simulink model "Grid_Forming_Inverters"  (R2024b)
settings: Solver=VariableStepAuto  StartTime=0.0  StopTime=GFM_Sim.t_stop  RelTol=1e-3
InitFcn:
  | addpath(genpath(fullfile(fileparts(fileparts(fileparts(get_param(bdroot,'FileName')))),'code','functions')));initialize_equipment_model_from_callback(bdroot);
undefined symbols (not defined in the file): Cf, f, GFM_CL, GFM_Droop, GFM_VI, GFM_VL, I_base_peak, L1, L2, Lg, R_C, R_L1, R_L2, Rg, S_base, V_base_phase, V_in, Vg
libraries: slpidlib x4, spsabctodq0Lib x4, spsThreePhaseSeriesRLCBranchLib x4, spsControlledVoltageSourceLib x3, spsCurrentMeasurementLib x3, spsVoltageMeasurementLib x3, spsGroundLib x2, spsThreePhaseVIMeasurementLib x2, spsdq0toabcLib x1, simulink x1, spsThreePhaseBreakerLib x1, spsThreePhaseProgrammableVoltageSourceLib x1
settings Model: Creator=ANYE  LastModifiedBy=AnYe
settings SolverCC: ZeroCrossAlgorithm=Adaptive
settings OptimizationCC: ReuseModelBlockBuffer=off
settings DebuggingCC: AlgebraicLoopMsg=none  IgnoredZcDiagnostic=none
settings RTWCC: GPUComputeCapability=3.5

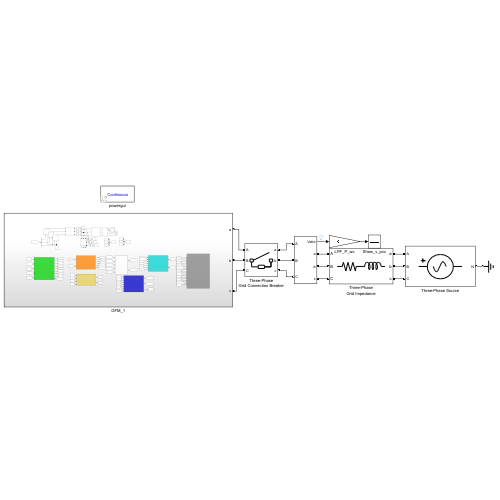
[thumbnail: Simulink's stored preview of the top-level diagram]
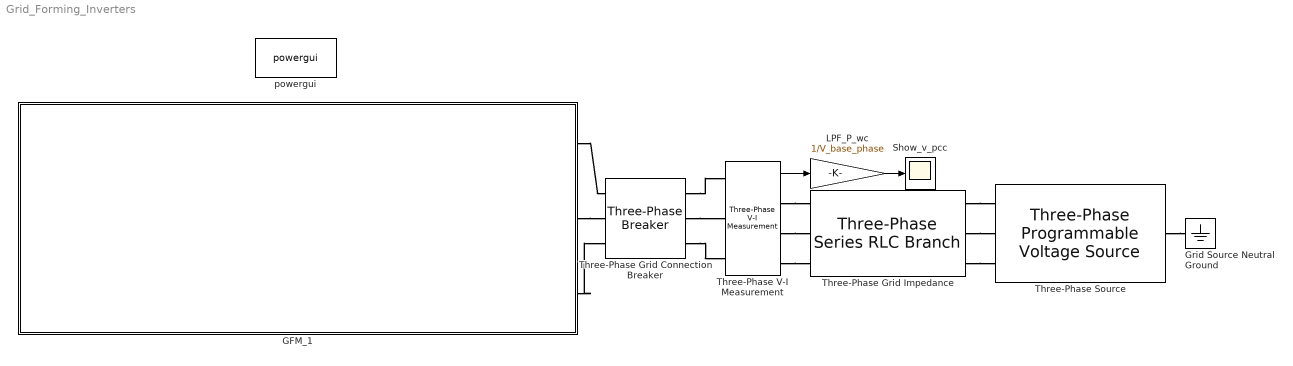
== system Grid_Forming_Inverters ==
  GFM_1 : Subsystem
  Grid Source Neutral Ground : spsGroundLib/Ground  LConnTagsString=a
  LPF_P_wc : Gain  Gain=1/V_base_phase
  Show_v_pcc : Scope
  Three-Phase Grid Connection Breaker : spsThreePhaseBreakerLib/Three-Phase Breaker  InitialState=open  SwitchA=on  SwitchB=on  SwitchC=on  SwitchTimes=t_close  External=off  BreakerResistance=0.01  SnubberResistance=1e6  SnubberCapacitance=inf  Measurements=None
  Three-Phase Grid Impedance : spsThreePhaseSeriesRLCBranchLib/Three-Phase Series RLC Branch  LConnTagsString=A|B|C  RConnTagsString=A|B|C  BranchType=RL  Resistance=Rg  Inductance=Lg  Capacitance=1e-6  Measurements=None
  Three-Phase V-I Measurement : spsThreePhaseVIMeasurementLib/Three-Phase V-I Measurement  VoltageMeasurement=phase-to-ground  SetLabelV=off  LabelV=Vabc  Vpu=off  VpuLL=off  CurrentMeasurement=no  SetLabelI=off  LabelI=Iabc  Ipu=off  Pbase=100e6  Vbase=500e3  OutputType=Complex  PhasorSimulation=off  PSBequivalent=0
  Three-Phase Source : spsThreePhaseProgrammableVoltageSourceLib/Three-Phase Programmable Voltage Source  PositiveSequence=[Vg 0 f]  VariationEntity=Amplitude  VariationType=Table of time-amplitude pairs  VariationTypeAlt=Step  VariationStep=0.5  VariationRate=10  VariationMagnitude=0.3  VariationFrequency=2  VariationTiming=[1 2]  VariationPhaseA=off  Amplitudes=GFM_GridSource.Amplitudes_pu  TimeValues=GFM_GridSource.TimeValues_s  HarmonicGeneration=off  HarmonicA=[3 0.2 -25 0]  HarmonicB=[2 0.15 35 2]  Timing="[0.05  3]"  BusType=swing  Pref=0  Qref=0  Qmin=-inf  Qmax=inf
  powergui : spspowerguiLib/powergui  Priority=1  SimulationMode=Continuous  SampleTime=50e-6  frequency=f  Iterations=50  frequencyindice=50  Pbase=100e6  ErrMax=1e-4  UnitsV=kV  UnitsW=MW  buscounter=0  FunctionMessages=off  echomessages=off  EnableUseOfTLC=off  CurrentSourceSwitches=off  DisableSnubberDevices=off  DisableRonSwitches=off  DisableVfSwitches=off  DisplayEquations=off  AutomaticDiscreteSolvers=off  SolverType=Tustin/Backward Euler (TBE)  Interpol=off  ExternalGateDelay=off  methode=off  Ts=100  x0status=blocks  SPID=on  SwTol=0  HookPort=off  NonlinearTolerance=1e-4  nMaxIteration=100  ContinueOnMaxIteration=off  RestoreLinks=warning  ResistiveCurrentMeasurement=off  Frange=[0:2:500]  Ylog=off  Xlog=on  ShowGrid=off  save=off  variable=ZData  structure=0  ZoomFFT=off  StartTime=0.0  cycles=1  DisplayStyle=1  fundamental=f  FreqAxis=off  MaxFrequency=1000  frequencyindicesteady=1  RmsSteady=1  display=off
  wires:
  Three-Phase V-I Measurement/1 -> LPF_P_wc/1
  LPF_P_wc/1 -> Show_v_pcc/1
  connections:
  Three-Phase V-I Measurement/RConn1 -- Three-Phase Grid Impedance/LConn1
  Three-Phase V-I Measurement/RConn2 -- Three-Phase Grid Impedance/LConn2
  Three-Phase V-I Measurement/RConn3 -- Three-Phase Grid Impedance/LConn3
  GFM_1/RConn1 -- Three-Phase Grid Connection Breaker/LConn1
  Three-Phase Grid Connection Breaker/RConn1 -- Three-Phase V-I Measurement/LConn1
  GFM_1/RConn2 -- Three-Phase Grid Connection Breaker/LConn2
  Three-Phase Grid Connection Breaker/RConn2 -- Three-Phase V-I Measurement/LConn2
  GFM_1/RConn3 -- Three-Phase Grid Connection Breaker/LConn3
  Three-Phase Grid Connection Breaker/RConn3 -- Three-Phase V-I Measurement/LConn3
  Three-Phase Grid Impedance/RConn1 -- Three-Phase Source/RConn1
  Three-Phase Grid Impedance/RConn2 -- Three-Phase Source/RConn2
  Three-Phase Grid Impedance/RConn3 -- Three-Phase Source/RConn3
  Three-Phase Source/LConn1 -- Grid Source Neutral Ground/LConn1

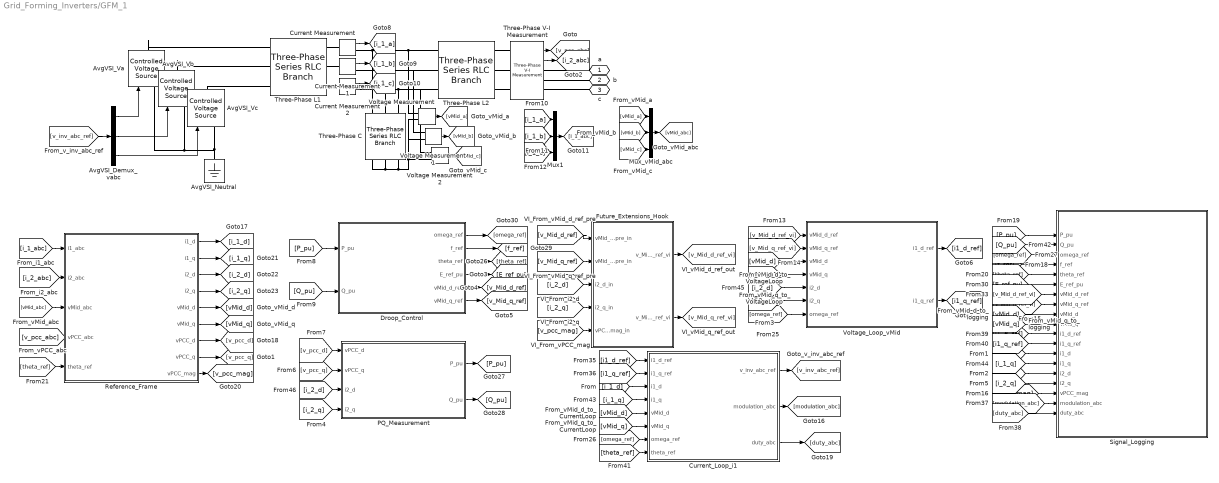
== system Grid_Forming_Inverters/GFM_1 ==
  AvgVSI_Demux_vabc : Demux  Outputs=3
  AvgVSI_Neutral : spsGroundLib/Ground  LConnTagsString=a
  AvgVSI_Va : spsControlledVoltageSourceLib/Controlled Voltage Source  Initialize=on  Source_Type=AC  Amplitude=0  Phase=0  Frequency=0  Measurements=None
  AvgVSI_Vb : spsControlledVoltageSourceLib/Controlled Voltage Source  Initialize=on  Source_Type=AC  Amplitude=0  Phase=0  Frequency=0  Measurements=None
  AvgVSI_Vc : spsControlledVoltageSourceLib/Controlled Voltage Source  Initialize=on  Source_Type=AC  Amplitude=0  Phase=0  Frequency=0  Measurements=None
  Current Measurement : spsCurrentMeasurementLib/Current Measurement  PhasorSimulation=off  OutputType=Complex  PSBequivalent=0
  Current Measurement1 : spsCurrentMeasurementLib/Current Measurement  PhasorSimulation=off  OutputType=Complex  PSBequivalent=0
  Current Measurement2 : spsCurrentMeasurementLib/Current Measurement  PhasorSimulation=off  OutputType=Complex  PSBequivalent=0
  Current_Loop_i1 : Subsystem
  Droop_Control : Subsystem
  Future_Extensions_Hook : Subsystem
      settings: AttributesFormatString=Unity pass-through in this version\nReserved: virtual impedance / LVRT / current limiting
  Mux1 : Mux  Inputs=3
  Mux_vMid_abc : Mux  Inputs=3
  PQ_Measurement : Subsystem
  Reference_Frame : Subsystem
  Signal_Logging : Subsystem
  Three-Phase C : spsThreePhaseSeriesRLCBranchLib/Three-Phase Series RLC Branch  LConnTagsString=A|B|C  RConnTagsString=A|B|C  BranchType=RC  Resistance=R_C  Inductance=1e-6  Capacitance=Cf  Measurements=None
  Three-Phase L1 : spsThreePhaseSeriesRLCBranchLib/Three-Phase Series RLC Branch  LConnTagsString=A|B|C  RConnTagsString=A|B|C  BranchType=RL  Resistance=R_L1  Inductance=L1  Capacitance=1e-6  Measurements=None
  Three-Phase L2 : spsThreePhaseSeriesRLCBranchLib/Three-Phase Series RLC Branch  LConnTagsString=A|B|C  RConnTagsString=A|B|C  BranchType=RL  Resistance=R_L2  Inductance=L2  Capacitance=1e-6  Measurements=None
  Three-Phase V-I Measurement : spsThreePhaseVIMeasurementLib/Three-Phase V-I Measurement  VoltageMeasurement=phase-to-ground  SetLabelV=off  LabelV=Vabc  Vpu=off  VpuLL=off  CurrentMeasurement=yes  SetLabelI=off  LabelI=Iabc  Ipu=off  Pbase=100e6  Vbase=500e3  OutputType=Complex  PhasorSimulation=off  PSBequivalent=0
  Voltage Measurement : spsVoltageMeasurementLib/Voltage Measurement  PhasorSimulation=off  OutputType=Complex  PSBequivalent=0
  Voltage Measurement1 : spsVoltageMeasurementLib/Voltage Measurement  PhasorSimulation=off  OutputType=Complex  PSBequivalent=0
  Voltage Measurement2 : spsVoltageMeasurementLib/Voltage Measurement  PhasorSimulation=off  OutputType=Complex  PSBequivalent=0
  Voltage_Loop_vMid : Subsystem
  a : PMIOPort  Side=Right
  b : PMIOPort  Port=2  Side=Right
  c : PMIOPort  Port=3  Side=Right
  wires:
  Three-Phase V-I Measurement/1 -> [v_pcc_abc]
  Current Measurement/1 -> [i_1_a]
  Current Measurement1/1 -> [i_1_b]
  Current Measurement2/1 -> [i_1_c]
  Voltage Measurement1/1 -> [vMid_b]
  Three-Phase V-I Measurement/2 -> [i_2_abc]
  Voltage Measurement2/1 -> [vMid_c]
  Voltage Measurement/1 -> [vMid_a]
  Mux_vMid_abc/1 -> [vMid_abc]
  Mux1/1 -> [i_1_abc]
  [i_1_c] -> Mux1/3
  [vMid_c] -> Mux_vMid_abc/3
  [vMid_b] -> Mux_vMid_abc/2
  [vMid_a] -> Mux_vMid_abc/1
  [i_1_a] -> Mux1/1
  [i_1_b] -> Mux1/2
  [v_inv_abc_ref] -> AvgVSI_Demux_vabc/1
  AvgVSI_Demux_vabc/1 -> AvgVSI_Va/1
  AvgVSI_Demux_vabc/2 -> AvgVSI_Vb/1
  AvgVSI_Demux_vabc/3 -> AvgVSI_Vc/1
  Current_Loop_i1/3(duty_abc) -> [duty_abc]
  Current_Loop_i1/2(modulation_abc) -> [modulation_abc]
  [i1_d_ref] -> Current_Loop_i1/1(i1_d_ref)
  [omega_ref] -> Current_Loop_i1/7(omega_ref)
  [duty_abc] -> Signal_Logging/19(duty_abc)
  PQ_Measurement/2(Q_pu) -> [Q_pu]
  [omega_ref] -> Voltage_Loop_vMid/7(omega_ref)
  [omega_ref] -> Signal_Logging/3(omega_ref)
  Reference_Frame/2(i1_q) -> [i_1_q]
  [Q_pu] -> Signal_Logging/2(Q_pu)
  [i_1_d] -> Current_Loop_i1/3(i1_d)
  Droop_Control/4(E_ref_pu) -> [E_ref_pu]
  Droop_Control/5(vMid_d_ref) -> [v_Mid_d_ref]
  [i_2_q] -> Voltage_Loop_vMid/6(i2_q)
  Reference_Frame/3(i2_d) -> [i_2_d]
  [vMid_d] -> Signal_Logging/9(vMid_d)
  [v_pcc_q] -> PQ_Measurement/2(vPCC_q)
  [P_pu] -> Signal_Logging/1(P_pu)
  [vMid_q] -> Signal_Logging/10(vMid_q)
  [v_Mid_d_ref_vi] -> Signal_Logging/7(vMid_d_ref)
  [i_2_d] -> PQ_Measurement/3(i2_d)
  [theta_ref] -> Current_Loop_i1/8(theta_ref)
  Reference_Frame/6(vMid_q) -> [vMid_q]
  [i_2_d] -> Signal_Logging/15(i2_d)
  [i1_d_ref] -> Signal_Logging/11(i1_d_ref)
  [i_1_q] -> Signal_Logging/14(i1_q)
  [E_ref_pu] -> Signal_Logging/6(E_ref_pu)
  [i_2_d] -> Voltage_Loop_vMid/5(i2_d)
  PQ_Measurement/1(P_pu) -> [P_pu]
  Droop_Control/3(theta_ref) -> [theta_ref]
  Reference_Frame/9(vPCC_mag) -> [v_pcc_mag]
  [f_ref] -> Signal_Logging/4(f_ref)
  [i_1_d] -> Signal_Logging/13(i1_d)
  Reference_Frame/7(vPCC_d) -> [v_pcc_d]
  Droop_Control/2(f_ref) -> [f_ref]
  [i_2_q] -> Signal_Logging/16(i2_q)
  [i_1_q] -> Current_Loop_i1/4(i1_q)
  [v_pcc_d] -> PQ_Measurement/1(vPCC_d)
  Reference_Frame/4(i2_q) -> [i_2_q]
  Droop_Control/1(omega_ref) -> [omega_ref]
  [i_2_q] -> PQ_Measurement/4(i2_q)
  [modulation_abc] -> Signal_Logging/18(modulation_abc)
  Reference_Frame/1(i1_d) -> [i_1_d]
  [i1_q_ref] -> Current_Loop_i1/2(i1_q_ref)
  [vMid_q] -> Voltage_Loop_vMid/4(vMid_q)
  [i1_q_ref] -> Signal_Logging/12(i1_q_ref)
  [vMid_d] -> Voltage_Loop_vMid/3(vMid_d)
  [P_pu] -> Droop_Control/1(P_pu)
  [Q_pu] -> Droop_Control/2(Q_pu)
  [theta_ref] -> Reference_Frame/5(theta_ref)
  [vMid_q] -> Current_Loop_i1/6(vMid_q)
  [vMid_d] -> Current_Loop_i1/5(vMid_d)
  Reference_Frame/5(vMid_d) -> [vMid_d]
  [v_pcc_mag] -> Signal_Logging/17(vPCC_mag)
  Reference_Frame/8(vPCC_q) -> [v_pcc_q]
  [theta_ref] -> Signal_Logging/5(theta_ref)
  Current_Loop_i1/1(v_inv_abc_ref) -> [v_inv_abc_ref]
  [i_1_abc] -> Reference_Frame/1(i1_abc)
  [i_2_abc] -> Reference_Frame/2(i2_abc)
  [vMid_abc] -> Reference_Frame/3(vMid_abc)
  [v_pcc_abc] -> Reference_Frame/4(vPCC_abc)
  [v_Mid_d_ref_vi] -> Voltage_Loop_vMid/1(vMid_d_ref)
  Droop_Control/6(vMid_q_ref) -> [v_Mid_q_ref]
  [v_Mid_q_ref_vi] -> Voltage_Loop_vMid/2(vMid_q_ref)
  [v_Mid_q_ref_vi] -> Signal_Logging/8(vMid_q_ref)
  [v_Mid_d_ref] -> Future_Extensions_Hook/1(vMid_d_ref_pre_in)
  [v_Mid_q_ref] -> Future_Extensions_Hook/2(vMid_q_ref_pre_in)
  [i_2_d] -> Future_Extensions_Hook/3(i2_d_in)
  [i_2_q] -> Future_Extensions_Hook/4(i2_q_in)
  Voltage_Loop_vMid/1(i1_d_ref) -> [i1_d_ref]
  Voltage_Loop_vMid/2(i1_q_ref) -> [i1_q_ref]
  Future_Extensions_Hook/2(v_Mid_q_ref_vi) -> [v_Mid_q_ref_vi]
  Future_Extensions_Hook/1(v_Mid_d_ref_vi) -> [v_Mid_d_ref_vi]
  [v_pcc_mag] -> Future_Extensions_Hook/5(vPCC_mag_in)
  connections:
  Current Measurement1/LConn1 -- Three-Phase L1/RConn2
  a/RConn1 -- Three-Phase V-I Measurement/RConn1
  Three-Phase C/RConn1 -- Voltage Measurement2/LConn2 -- Voltage Measurement1/LConn2 -- Voltage Measurement/LConn2 -- Three-Phase C/RConn3 -- Three-Phase C/RConn2
  Three-Phase C/LConn2 -- Three-Phase L2/LConn2 -- Voltage Measurement1/LConn1 -- Current Measurement1/RConn1
  Three-Phase C/LConn3 -- Three-Phase L2/LConn3 -- Voltage Measurement2/LConn1 -- Current Measurement2/RConn1
  Three-Phase V-I Measurement/LConn2 -- Three-Phase L2/RConn2
  Three-Phase C/LConn1 -- Current Measurement/RConn1 -- Three-Phase L2/LConn1 -- Voltage Measurement/LConn1
  Three-Phase L1/RConn3 -- Current Measurement2/LConn1
  Current Measurement/LConn1 -- Three-Phase L1/RConn1
  Three-Phase V-I Measurement/LConn3 -- Three-Phase L2/RConn3
  b/RConn1 -- Three-Phase V-I Measurement/RConn2
  Three-Phase V-I Measurement/LConn1 -- Three-Phase L2/RConn1
  c/RConn1 -- Three-Phase V-I Measurement/RConn3
  AvgVSI_Vb/RConn1 -- Three-Phase L1/LConn2
  AvgVSI_Va/RConn1 -- Three-Phase L1/LConn1
  Three-Phase L1/LConn3 -- AvgVSI_Vc/RConn1
  AvgVSI_Va/LConn1 -- AvgVSI_Vc/LConn1 -- AvgVSI_Neutral/LConn1 -- AvgVSI_Vb/LConn1

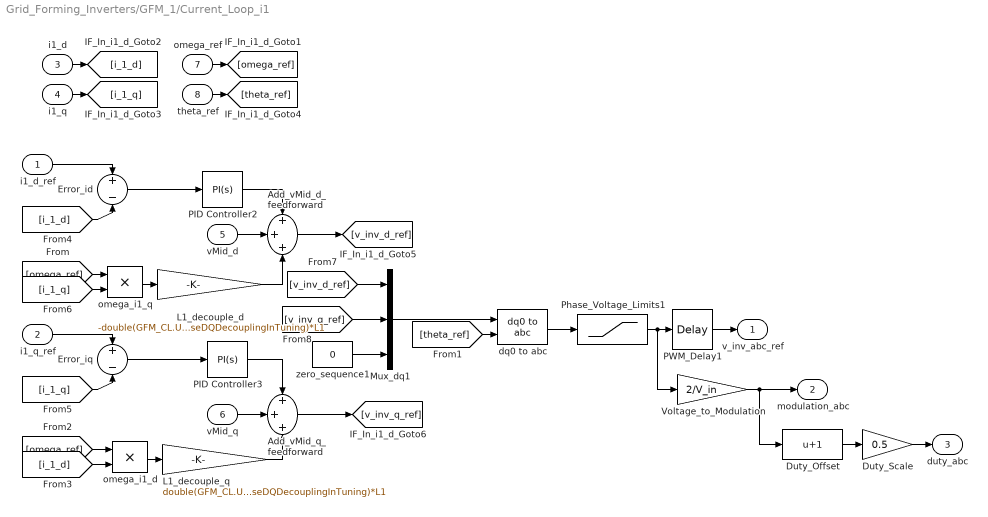
== system Grid_Forming_Inverters/GFM_1/Current_Loop_i1 ==
  i1_d_ref : Inport
  i1_q_ref : Inport  Port=2
  i1_d : Inport  Port=3
  i1_q : Inport  Port=4
  vMid_d : Inport  Port=5
  vMid_q : Inport  Port=6
  omega_ref : Inport  Port=7
  theta_ref : Inport  Port=8
  Add_vMid_d_feedforward : Sum  Inputs=+++
  Add_vMid_q_feedforward : Sum  Inputs=+++
  Duty_Offset : Bias  Bias=1  SaturateOnIntegerOverflow=off
  Duty_Scale : Gain  Gain=0.5
  Error_id : Sum  Inputs=+-
  Error_iq : Sum  Inputs=+-
  L1_decouple_d : Gain  Gain=-double(GFM_CL.UseDQDecouplingInTuning)*L1
  L1_decouple_q : Gain  Gain=double(GFM_CL.UseDQDecouplingInTuning)*L1
  Mux_dq1 : Mux  Inputs=3
  PID Controller2 : slpidlib/PID Controller  Controller=PI  Form=Parallel  TimeDomain=Continuous-time  UseExternalTs=off  SampleTime=-1  IntegratorMethod=Forward Euler  FilterMethod=Forward Euler  ControllerParametersSource=internal  P=GFM_CL.Kp  I=GFM_CL.Ki  UseKiTs=off  D=0  UseExternalDerivativeSource=off  N=100  UseFilter=on  TunerSelectOption=Transfer Function Based (PID Tuner App)  InitialConditionSource=internal  InitialConditionForIntegrator=0  InitialConditionForFilter=0  DifferentiatorICPrevScaledInput=0  ExternalReset=none  TrackingMode=off  Kt=1  LimitOutput=off  SatLimitsSource=internal  UpperSaturationLimit=inf  LowerSaturationLimit=-inf  LinearizeAsGain=on  AntiWindupMode=none  Kb=1  LimitIntegrator=off  UpperIntegratorSaturationLimit=inf  LowerIntegratorSaturationLimit=-inf  POutMin=[]  POutMax=[]  IOutMin=[]  IOutMax=[]  DOutMin=[]  DOutMax=[]  NOutMin=[]  NOutMax=[]  SumOutMin=[]  SumOutMax=[]  SaturationOutMin=[]  SaturationOutMax=[]  PParamMin=[]  PParamMax=[]  IParamMin=[]  IParamMax=[]  DParamMin=[]  DParamMax=[]  NParamMin=[]  NParamMax=[]  KbParamMin=[]  KbParamMax=[]  KtParamMin=[]  KtParamMax=[]  KbOutMin=[]  KbOutMax=[]  KtOutMin=[]  KtOutMax=[]  IntegratorOutMin=[]  IntegratorOutMax=[]  FilterOutMin=[]  FilterOutMax=[]  SumI1OutMin=[]  SumI1OutMax=[]  SumI2OutMin=[]  SumI2OutMax=[]  SumI3OutMin=[]  SumI3OutMax=[]  SumI4OutMin=[]  SumI4OutMax=[]  SumDOutMin=[]  SumDOutMax=[]  DifferentiatorOutMin=[]  DifferentiatorOutMax=[]  FilterDiffOutCoefMin=[]  FilterDiffOutCoefMax=[]  ReciprocalOutMin=[]  ReciprocalOutMax=[]  SumDenOutMin=[]  SumDenOutMax=[]  SumNumOutMin=[]  SumNumOutMax=[]  DivideOutMin=[]  DivideOutMax=[]  UdiffTsProdOutMin=[]  UdiffTsProdOutMax=[]  NTsProdOutMin=[]  NTsProdOutMax=[]  UintegralTsProdOutMin=[]  UintegralTsProdOutMax=[]  UngainTsProdOutMin=[]  UngainTsProdOutMax=[]  ClampingZeroOutDataTypeStr=Inherit: Inherit via back propagation  ClampingZeroOutMin=[]  ClampingZeroOutMax=[]  FilterDenConstantOutDataTypeStr=Inherit: Inherit via back propagation  FilterDenConstantOutMin=[]  FilterDenConstantOutMax=[]  PCopyOutDataTypeStr=Inherit: Inherit via back propagation  PCopyOutMin=[]  PCopyOutMax=[]  NCopyOutDataTypeStr=Inherit: Inherit via back propagation  NCopyOutMin=[]  NCopyOutMax=[]  IntegratorContinuousStateAttributes=''  IntegratorStateMustResolveToSignalObject=off  IntegratorRTWStateStorageClass=Auto  FilterContinuousStateAttributes=''  FilterStateMustResolveToSignalObject=off  FilterRTWStateStorageClass=Auto  ParallelPVariant=InternalParameters  IdealPVariant=Disabled  IVariant=InternalParameters  DVariant=Disabled  IntegratorVariant=Continuous  SatVariant=Disabled  AWVariant=Passthrough  PCopyVariant=Disabled  TRVariant=Disabled  FdbkBlocksVariant=Forward  IdealPFdbkVariant=Disabled  SatFdbkVariant=Disabled  DerivativeFilterVariant=Disabled  NVariant=Disabled  NCopyVariant=Disabled_SignalSpec  FilterICVariant=Disabled  IntegratorICVariant=InternalICs  ExternalResetVariant=Disabled  TRSumVariant=Passthrough  SumFdbkVariant=Disabled  SumVariant=Sum_PI  TsampFilterVariant=InternalTs  TsampNgainVariant=Passthrough  TsampIntegralVariant=Disabled_SignalSpec  ExternalSaturationOutDataTypeStr=Inherit: Same as second input  DerivativeSourceVariant=Disabled  PreIntVariant=InternalPreInt
  PID Controller3 : slpidlib/PID Controller  Controller=PI  Form=Parallel  TimeDomain=Continuous-time  UseExternalTs=off  SampleTime=-1  IntegratorMethod=Forward Euler  FilterMethod=Forward Euler  ControllerParametersSource=internal  P=GFM_CL.Kp  I=GFM_CL.Ki  UseKiTs=off  D=0  UseExternalDerivativeSource=off  N=100  UseFilter=on  TunerSelectOption=Transfer Function Based (PID Tuner App)  InitialConditionSource=internal  InitialConditionForIntegrator=0  InitialConditionForFilter=0  DifferentiatorICPrevScaledInput=0  ExternalReset=none  TrackingMode=off  Kt=1  LimitOutput=off  SatLimitsSource=internal  UpperSaturationLimit=inf  LowerSaturationLimit=-inf  LinearizeAsGain=on  AntiWindupMode=none  Kb=1  LimitIntegrator=off  UpperIntegratorSaturationLimit=inf  LowerIntegratorSaturationLimit=-inf  POutMin=[]  POutMax=[]  IOutMin=[]  IOutMax=[]  DOutMin=[]  DOutMax=[]  NOutMin=[]  NOutMax=[]  SumOutMin=[]  SumOutMax=[]  SaturationOutMin=[]  SaturationOutMax=[]  PParamMin=[]  PParamMax=[]  IParamMin=[]  IParamMax=[]  DParamMin=[]  DParamMax=[]  NParamMin=[]  NParamMax=[]  KbParamMin=[]  KbParamMax=[]  KtParamMin=[]  KtParamMax=[]  KbOutMin=[]  KbOutMax=[]  KtOutMin=[]  KtOutMax=[]  IntegratorOutMin=[]  IntegratorOutMax=[]  FilterOutMin=[]  FilterOutMax=[]  SumI1OutMin=[]  SumI1OutMax=[]  SumI2OutMin=[]  SumI2OutMax=[]  SumI3OutMin=[]  SumI3OutMax=[]  SumI4OutMin=[]  SumI4OutMax=[]  SumDOutMin=[]  SumDOutMax=[]  DifferentiatorOutMin=[]  DifferentiatorOutMax=[]  FilterDiffOutCoefMin=[]  FilterDiffOutCoefMax=[]  ReciprocalOutMin=[]  ReciprocalOutMax=[]  SumDenOutMin=[]  SumDenOutMax=[]  SumNumOutMin=[]  SumNumOutMax=[]  DivideOutMin=[]  DivideOutMax=[]  UdiffTsProdOutMin=[]  UdiffTsProdOutMax=[]  NTsProdOutMin=[]  NTsProdOutMax=[]  UintegralTsProdOutMin=[]  UintegralTsProdOutMax=[]  UngainTsProdOutMin=[]  UngainTsProdOutMax=[]  ClampingZeroOutDataTypeStr=Inherit: Inherit via back propagation  ClampingZeroOutMin=[]  ClampingZeroOutMax=[]  FilterDenConstantOutDataTypeStr=Inherit: Inherit via back propagation  FilterDenConstantOutMin=[]  FilterDenConstantOutMax=[]  PCopyOutDataTypeStr=Inherit: Inherit via back propagation  PCopyOutMin=[]  PCopyOutMax=[]  NCopyOutDataTypeStr=Inherit: Inherit via back propagation  NCopyOutMin=[]  NCopyOutMax=[]  IntegratorContinuousStateAttributes=''  IntegratorStateMustResolveToSignalObject=off  IntegratorRTWStateStorageClass=Auto  FilterContinuousStateAttributes=''  FilterStateMustResolveToSignalObject=off  FilterRTWStateStorageClass=Auto  ParallelPVariant=InternalParameters  IdealPVariant=Disabled  IVariant=InternalParameters  DVariant=Disabled  IntegratorVariant=Continuous  SatVariant=Disabled  AWVariant=Passthrough  PCopyVariant=Disabled  TRVariant=Disabled  FdbkBlocksVariant=Forward  IdealPFdbkVariant=Disabled  SatFdbkVariant=Disabled  DerivativeFilterVariant=Disabled  NVariant=Disabled  NCopyVariant=Disabled_SignalSpec  FilterICVariant=Disabled  IntegratorICVariant=InternalICs  ExternalResetVariant=Disabled  TRSumVariant=Passthrough  SumFdbkVariant=Disabled  SumVariant=Sum_PI  TsampFilterVariant=InternalTs  TsampNgainVariant=Passthrough  TsampIntegralVariant=Disabled_SignalSpec  ExternalSaturationOutDataTypeStr=Inherit: Same as second input  DerivativeSourceVariant=Disabled  PreIntVariant=InternalPreInt
  PWM_Delay1 : TransportDelay  DelayTime=GFM_CL.PWMDelay
  Phase_Voltage_Limits1 : Saturate  UpperLimit=V_in/2  LowerLimit=-V_in/2
  Voltage_to_Modulation : Gain  Gain=2/V_in
  dq0 to abc : spsdq0toabcLib/dq0 to abc  Alignment=Aligned with phase A axis
  omega_i1_d : Product
  omega_i1_q : Product
  zero_sequence1 : Constant  Value=0
  v_inv_abc_ref : Outport
  modulation_abc : Outport  Port=2
  duty_abc : Outport  Port=3
  wires:
  i1_d_ref/1 -> Error_id/1
  i1_q_ref/1 -> Error_iq/1
  omega_i1_q/1 -> L1_decouple_d/1
  omega_i1_d/1 -> L1_decouple_q/1
  vMid_d/1 -> Add_vMid_d_feedforward/2
  L1_decouple_d/1 -> Add_vMid_d_feedforward/3
  vMid_q/1 -> Add_vMid_q_feedforward/2
  L1_decouple_q/1 -> Add_vMid_q_feedforward/3
  Add_vMid_d_feedforward/1 -> [v_inv_d_ref]
  Add_vMid_q_feedforward/1 -> [v_inv_q_ref]
  omega_ref/1 -> [omega_ref]
  [omega_ref] -> omega_i1_q/1
  [omega_ref] -> omega_i1_d/1
  [i_1_d] -> omega_i1_d/2
  i1_d/1 -> [i_1_d]
  [i_1_d] -> Error_id/2
  i1_q/1 -> [i_1_q]
  [i_1_q] -> Error_iq/2
  [i_1_q] -> omega_i1_q/2
  PID Controller2/1 -> Add_vMid_d_feedforward/1
  Error_id/1 -> PID Controller2/1
  Error_iq/1 -> PID Controller3/1
  PID Controller3/1 -> Add_vMid_q_feedforward/1
  [theta_ref] -> dq0 to abc/2
  theta_ref/1 -> [theta_ref]
  Mux_dq1/1 -> dq0 to abc/1
  zero_sequence1/1 -> Mux_dq1/3
  [v_inv_q_ref] -> Mux_dq1/2
  [v_inv_d_ref] -> Mux_dq1/1
  Phase_Voltage_Limits1/1 -> Voltage_to_Modulation/1, PWM_Delay1/1
  dq0 to abc/1 -> Phase_Voltage_Limits1/1
  PWM_Delay1/1 -> v_inv_abc_ref/1
  Duty_Offset/1 -> Duty_Scale/1
  Duty_Scale/1 -> duty_abc/1
  Voltage_to_Modulation/1 -> modulation_abc/1, Duty_Offset/1

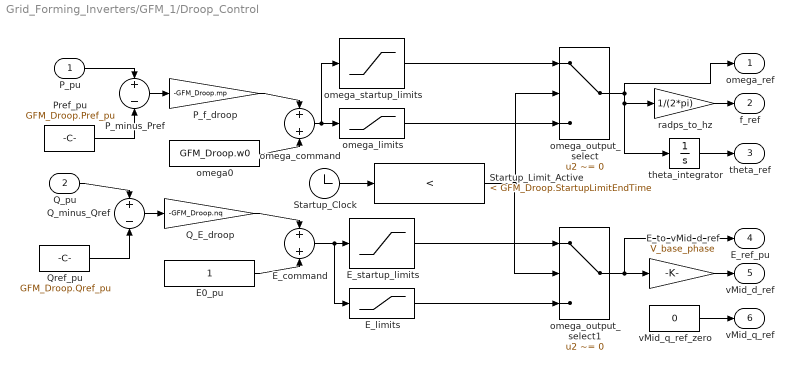
== system Grid_Forming_Inverters/GFM_1/Droop_Control ==
  P_pu : Inport
  Q_pu : Inport  Port=2
  E0_pu : Constant
  E_command : Sum
  E_limits : Saturate  UpperLimit=GFM_Droop.E_max_pu  LowerLimit=GFM_Droop.E_min_pu
  E_startup_limits : Saturate  UpperLimit=GFM_Droop.Startup_E_max_pu  LowerLimit=GFM_Droop.Startup_E_min_pu
  E_to_vMid_d_ref : Gain  Gain=V_base_phase
  P_f_droop : Gain  Gain=-GFM_Droop.mp
  P_minus_Pref : Sum  Inputs=+-
  Pref_pu : Constant  Value=GFM_Droop.Pref_pu
  Q_E_droop : Gain  Gain=-GFM_Droop.nq
  Q_minus_Qref : Sum  Inputs=+-
  Qref_pu : Constant  Value=GFM_Droop.Qref_pu
  Startup_Clock : Clock
  Startup_Limit_Active : simulink/Logic and Bit Operations/Compare To Constant  relop=<  const=GFM_Droop.StartupLimitEndTime  OutDataTypeStr=boolean
  omega0 : Constant  Value=GFM_Droop.w0
  omega_command : Sum
  omega_limits : Saturate  UpperLimit=GFM_Droop.w_max  LowerLimit=GFM_Droop.w_min
  omega_output_select : Switch  Criteria=u2 ~= 0  SaturateOnIntegerOverflow=off  InputSameDT=off
  omega_output_select1 : Switch  Criteria=u2 ~= 0  SaturateOnIntegerOverflow=off  InputSameDT=off
  omega_startup_limits : Saturate  UpperLimit=GFM_Droop.Startup_w_max  LowerLimit=GFM_Droop.Startup_w_min
  radps_to_hz : Gain  Gain=1/(2*pi)
  theta_integrator : Integrator  InitialCondition=GFM_Droop.theta0
  vMid_q_ref_zero : Constant  Value=0
  omega_ref : Outport
  f_ref : Outport  Port=2
  theta_ref : Outport  Port=3
  E_ref_pu : Outport  Port=4
  vMid_d_ref : Outport  Port=5
  vMid_q_ref : Outport  Port=6
  wires:
  P_pu/1 -> P_minus_Pref/1
  Pref_pu/1 -> P_minus_Pref/2
  P_minus_Pref/1 -> P_f_droop/1
  P_f_droop/1 -> omega_command/1
  omega0/1 -> omega_command/2
  omega_command/1 -> omega_limits/1, omega_startup_limits/1
  radps_to_hz/1 -> f_ref/1
  theta_integrator/1 -> theta_ref/1
  Q_pu/1 -> Q_minus_Qref/1
  Qref_pu/1 -> Q_minus_Qref/2
  Q_minus_Qref/1 -> Q_E_droop/1
  Q_E_droop/1 -> E_command/1
  E0_pu/1 -> E_command/2
  E_command/1 -> E_limits/1, E_startup_limits/1
  E_to_vMid_d_ref/1 -> vMid_d_ref/1
  vMid_q_ref_zero/1 -> vMid_q_ref/1
  omega_limits/1 -> omega_output_select/3
  omega_startup_limits/1 -> omega_output_select/1
  omega_output_select/1 -> radps_to_hz/1, theta_integrator/1, omega_ref/1
  Startup_Clock/1 -> Startup_Limit_Active/1
  Startup_Limit_Active/1 -> omega_output_select1/2, omega_output_select/2
  E_limits/1 -> omega_output_select1/3
  E_startup_limits/1 -> omega_output_select1/1
  omega_output_select1/1 -> E_to_vMid_d_ref/1, E_ref_pu/1

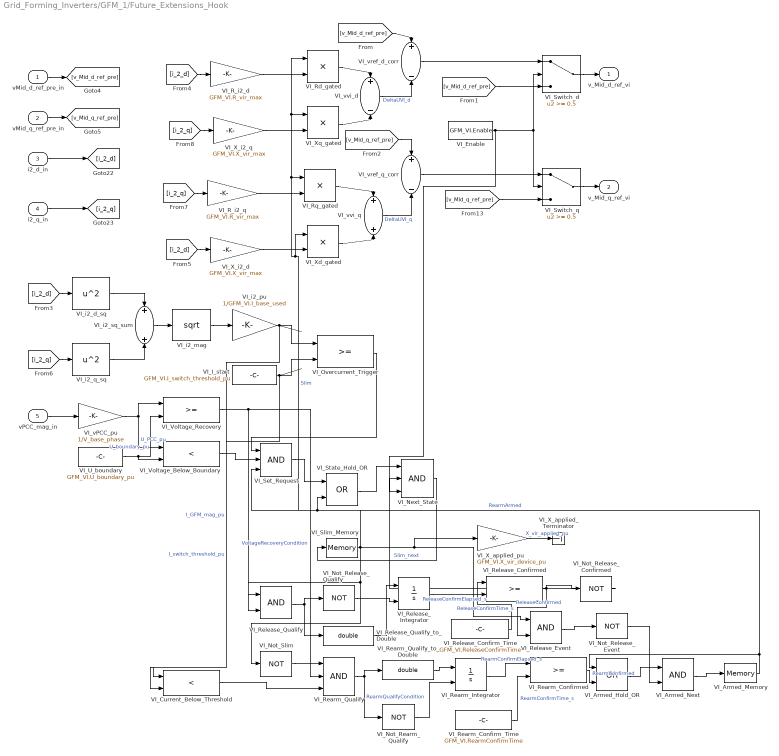
== system Grid_Forming_Inverters/GFM_1/Future_Extensions_Hook ==
  vMid_d_ref_pre_in : Inport
  vMid_q_ref_pre_in : Inport  Port=2
  i2_d_in : Inport  Port=3
  i2_q_in : Inport  Port=4
  vPCC_mag_in : Inport  Port=5
  VI_Armed_Hold_OR : Logic  Operator=OR  AllPortsSameDT=off  OutDataTypeStr=boolean
  VI_Armed_Memory : Memory  InitialCondition=1
  VI_Armed_Next : Logic  AllPortsSameDT=off  OutDataTypeStr=boolean
  VI_Current_Below_Threshold : RelationalOperator  Operator=<  OutDataTypeStr=boolean  RndMeth=Simplest  InputSameDT=off
  VI_Enable : Constant  Value=GFM_VI.Enable
  VI_I_start : Constant  Value=GFM_VI.I_switch_threshold_pu
  VI_Next_State : Logic  Inputs=3  AllPortsSameDT=off  OutDataTypeStr=boolean
  VI_Not_Rearm_Qualify : Logic  Operator=NOT  AllPortsSameDT=off  OutDataTypeStr=boolean
  VI_Not_Release_Confirmed : Logic  Operator=NOT  AllPortsSameDT=off  OutDataTypeStr=boolean
  VI_Not_Release_Event : Logic  Operator=NOT  AllPortsSameDT=off  OutDataTypeStr=boolean
  VI_Not_Release_Qualify : Logic  Operator=NOT  AllPortsSameDT=off  OutDataTypeStr=boolean
  VI_Not_Slim : Logic  Operator=NOT  AllPortsSameDT=off  OutDataTypeStr=boolean
  VI_Overcurrent_Trigger : RelationalOperator  OutDataTypeStr=boolean  RndMeth=Simplest  InputSameDT=off
  VI_R_i2_d : Gain  Gain=GFM_VI.R_vir_max
  VI_R_i2_q : Gain  Gain=GFM_VI.R_vir_max
  VI_Rd_gated : Product  Inputs=**
  VI_Rearm_Confirm_Time : Constant  Value=GFM_VI.RearmConfirmTime
  VI_Rearm_Confirmed : RelationalOperator  OutDataTypeStr=boolean  RndMeth=Simplest  InputSameDT=off
  VI_Rearm_Integrator : Integrator  ExternalReset=level  LimitOutput=on  UpperSaturationLimit=GFM_VI.RearmConfirmTime  LowerSaturationLimit=0
  VI_Rearm_Qualify : Logic  Inputs=3  AllPortsSameDT=off  OutDataTypeStr=boolean
  VI_Rearm_Qualify_to_Double : DataTypeConversion  OutDataTypeStr=double  SaturateOnIntegerOverflow=off  RndMeth=Floor
  VI_Release_Confirm_Time : Constant  Value=GFM_VI.ReleaseConfirmTime
  VI_Release_Confirmed : RelationalOperator  OutDataTypeStr=boolean  RndMeth=Simplest  InputSameDT=off
  VI_Release_Event : Logic  AllPortsSameDT=off  OutDataTypeStr=boolean
  VI_Release_Integrator : Integrator  ExternalReset=level  LimitOutput=on  UpperSaturationLimit=GFM_VI.ReleaseConfirmTime  LowerSaturationLimit=0
  VI_Release_Qualify : Logic  AllPortsSameDT=off  OutDataTypeStr=boolean
  VI_Release_Qualify_to_Double : DataTypeConversion  OutDataTypeStr=double  SaturateOnIntegerOverflow=off  RndMeth=Floor
  VI_Rq_gated : Product  Inputs=**
  VI_Set_Request : Logic  Inputs=3  AllPortsSameDT=off  OutDataTypeStr=boolean
  VI_Slim_Memory : Memory
  VI_State_Hold_OR : Logic  Operator=OR  AllPortsSameDT=off  OutDataTypeStr=boolean
  VI_Switch_d : Switch  Threshold=0.5  SaturateOnIntegerOverflow=off  InputSameDT=off
  VI_Switch_q : Switch  Threshold=0.5  SaturateOnIntegerOverflow=off  InputSameDT=off
  VI_U_boundary : Constant  Value=GFM_VI.U_boundary_pu
  VI_Voltage_Below_Boundary : RelationalOperator  Operator=<  OutDataTypeStr=boolean  RndMeth=Simplest  InputSameDT=off
  VI_Voltage_Recovery : RelationalOperator  OutDataTypeStr=boolean  RndMeth=Simplest  InputSameDT=off
  VI_X_applied_Terminator : Terminator
  VI_X_applied_pu : Gain  Gain=GFM_VI.X_vir_device_pu  ParamDataTypeStr=double  OutDataTypeStr=double
  VI_X_i2_d : Gain  Gain=GFM_VI.X_vir_max
  VI_X_i2_q : Gain  Gain=GFM_VI.X_vir_max
  VI_Xd_gated : Product  Inputs=**
  VI_Xq_gated : Product  Inputs=**
  VI_i2_d_sq : Math  Operator=square
  VI_i2_mag : Math  Operator=sqrt
  VI_i2_pu : Gain  Gain=1/GFM_VI.I_base_used
  VI_i2_q_sq : Math  Operator=square
  VI_i2_sq_sum : Sum
  VI_vPCC_pu : Gain  Gain=1/V_base_phase
  VI_vref_d_corr : Sum  Inputs=+-
  VI_vref_q_corr : Sum  Inputs=+-
  VI_vvi_d : Sum  Inputs=+-
  VI_vvi_q : Sum
  v_Mid_d_ref_vi : Outport
  v_Mid_q_ref_vi : Outport  Port=2
  wires:
  VI_i2_d_sq/1 -> VI_i2_sq_sum/1
  VI_i2_q_sq/1 -> VI_i2_sq_sum/2
  VI_i2_sq_sum/1 -> VI_i2_mag/1
  VI_i2_mag/1 -> VI_i2_pu/1
  VI_i2_pu/1 -> VI_Overcurrent_Trigger/1, VI_Current_Below_Threshold/1  "I_GFM_mag_pu"
  VI_I_start/1 -> VI_Overcurrent_Trigger/2, VI_Current_Below_Threshold/2  "I_switch_threshold_pu"
  ? -> ?
  VI_R_i2_d/1 -> VI_Rd_gated/2
  VI_R_i2_q/1 -> VI_Rq_gated/2
  VI_X_i2_d/1 -> VI_Xd_gated/2
  VI_X_i2_q/1 -> VI_Xq_gated/2
  VI_Rd_gated/1 -> VI_vvi_d/1
  VI_Xq_gated/1 -> VI_vvi_d/2
  VI_Rq_gated/1 -> VI_vvi_q/1
  VI_Xd_gated/1 -> VI_vvi_q/2
  VI_vvi_d/1 -> VI_vref_d_corr/2  "DeltaUVI_d"
  VI_vvi_q/1 -> VI_vref_q_corr/2  "DeltaUVI_q"
  VI_vref_d_corr/1 -> VI_Switch_d/1
  VI_Enable/1 -> VI_Switch_d/2, VI_Switch_q/2, VI_Next_State/3
  VI_vref_q_corr/1 -> VI_Switch_q/1
  VI_Switch_d/1 -> v_Mid_d_ref_vi/1
  VI_Switch_q/1 -> v_Mid_q_ref_vi/1
  vMid_d_ref_pre_in/1 -> [v_Mid_d_ref_pre]
  [v_Mid_d_ref_pre] -> VI_vref_d_corr/1
  [v_Mid_d_ref_pre] -> VI_Switch_d/3
  vMid_q_ref_pre_in/1 -> [v_Mid_q_ref_pre]
  [v_Mid_q_ref_pre] -> VI_vref_q_corr/1
  i2_d_in/1 -> [i_2_d]
  [i_2_d] -> VI_i2_d_sq/1
  [i_2_d] -> VI_R_i2_d/1
  [i_2_d] -> VI_X_i2_d/1
  i2_q_in/1 -> [i_2_q]
  [i_2_q] -> VI_i2_q_sq/1
  [i_2_q] -> VI_X_i2_q/1
  [i_2_q] -> VI_R_i2_q/1
  [v_Mid_q_ref_pre] -> VI_Switch_q/3
  vPCC_mag_in/1 -> VI_vPCC_pu/1
  VI_vPCC_pu/1 -> VI_Voltage_Recovery/1, VI_Voltage_Below_Boundary/1  "U_PCC_pu"
  VI_U_boundary/1 -> VI_Voltage_Recovery/2, VI_Voltage_Below_Boundary/2  "U_boundary_pu"
  VI_Overcurrent_Trigger/1 -> VI_Set_Request/1
  VI_Voltage_Below_Boundary/1 -> VI_Set_Request/2
  VI_Set_Request/1 -> VI_State_Hold_OR/1
  VI_Slim_Memory/1 -> VI_Release_Qualify/2, VI_Not_Slim/1, VI_X_applied_pu/1, VI_Release_Event/1, VI_Rd_gated/1, VI_Xq_gated/1, VI_Rq_gated/1, VI_Xd_gated/1, VI_State_Hold_OR/2  "Slim"
  VI_State_Hold_OR/1 -> VI_Next_State/1
  VI_Not_Release_Confirmed/1 -> VI_Next_State/2
  VI_X_applied_pu/1 -> VI_X_applied_Terminator/1  "X_vir_applied_pu"
  VI_Next_State/1 -> VI_Slim_Memory/1  "Slim_next"
  VI_Voltage_Recovery/1 -> VI_Release_Qualify/1, VI_Rearm_Qualify/2  "VoltageRecoveryCondition"
  VI_Release_Qualify/1 -> VI_Release_Qualify_to_Double/1, VI_Not_Release_Qualify/1
  VI_Release_Qualify_to_Double/1 -> VI_Release_Integrator/1
  VI_Not_Release_Qualify/1 -> VI_Release_Integrator/2
  VI_Release_Integrator/1 -> VI_Release_Confirmed/1  "ReleaseConfirmElapsed_s"
  VI_Release_Confirm_Time/1 -> VI_Release_Confirmed/2  "ReleaseConfirmTime_s"
  VI_Release_Confirmed/1 -> VI_Not_Release_Confirmed/1, VI_Release_Event/2  "ReleaseConfirmed"
  VI_Not_Slim/1 -> VI_Rearm_Qualify/1
  VI_Current_Below_Threshold/1 -> VI_Rearm_Qualify/3
  VI_Rearm_Qualify/1 -> VI_Rearm_Qualify_to_Double/1, VI_Not_Rearm_Qualify/1  "RearmQualifyCondition"
  VI_Rearm_Qualify_to_Double/1 -> VI_Rearm_Integrator/1
  VI_Not_Rearm_Qualify/1 -> VI_Rearm_Integrator/2
  VI_Rearm_Integrator/1 -> VI_Rearm_Confirmed/1  "RearmConfirmElapsed_s"
  VI_Rearm_Confirm_Time/1 -> VI_Rearm_Confirmed/2  "RearmConfirmTime_s"
  VI_Release_Event/1 -> VI_Not_Release_Event/1
  VI_Armed_Memory/1 -> VI_Armed_Hold_OR/1, VI_Set_Request/3  "RearmArmed"
  VI_Rearm_Confirmed/1 -> VI_Armed_Hold_OR/2  "RearmConfirmed"
  VI_Armed_Hold_OR/1 -> VI_Armed_Next/1
  VI_Not_Release_Event/1 -> VI_Armed_Next/2
  VI_Armed_Next/1 -> VI_Armed_Memory/1

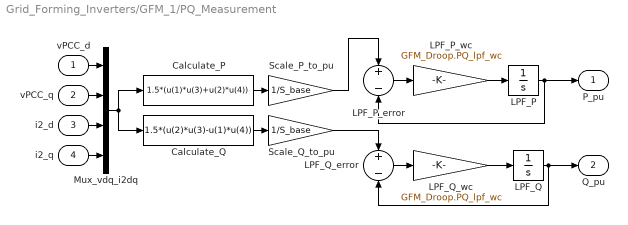
== system Grid_Forming_Inverters/GFM_1/PQ_Measurement ==
  vPCC_d : Inport
  vPCC_q : Inport  Port=2
  i2_d : Inport  Port=3
  i2_q : Inport  Port=4
  Calculate_P : Fcn  Expr=1.5*(u(1)*u(3)+u(2)*u(4))
  Calculate_Q : Fcn  Expr=1.5*(u(2)*u(3)-u(1)*u(4))
  LPF_P : Integrator  InitialCondition=GFM_Droop.Pref_pu
  LPF_P_error : Sum  Inputs=+-
  LPF_P_wc : Gain  Gain=GFM_Droop.PQ_lpf_wc
  LPF_Q : Integrator  InitialCondition=GFM_Droop.Qref_pu
  LPF_Q_error : Sum  Inputs=+-
  LPF_Q_wc : Gain  Gain=GFM_Droop.PQ_lpf_wc
  Mux_vdq_i2dq : Mux
  Scale_P_to_pu : Gain  Gain=1/S_base
  Scale_Q_to_pu : Gain  Gain=1/S_base
  P_pu : Outport
  Q_pu : Outport  Port=2
  wires:
  vPCC_d/1 -> Mux_vdq_i2dq/1
  vPCC_q/1 -> Mux_vdq_i2dq/2
  i2_d/1 -> Mux_vdq_i2dq/3
  i2_q/1 -> Mux_vdq_i2dq/4
  Mux_vdq_i2dq/1 -> Calculate_P/1, Calculate_Q/1
  Calculate_P/1 -> Scale_P_to_pu/1
  Scale_P_to_pu/1 -> LPF_P_error/1
  LPF_P/1 -> P_pu/1, LPF_P_error/2
  LPF_P_error/1 -> LPF_P_wc/1
  LPF_P_wc/1 -> LPF_P/1
  Calculate_Q/1 -> Scale_Q_to_pu/1
  Scale_Q_to_pu/1 -> LPF_Q_error/1
  LPF_Q/1 -> LPF_Q_error/2, Q_pu/1
  LPF_Q_error/1 -> LPF_Q_wc/1
  LPF_Q_wc/1 -> LPF_Q/1

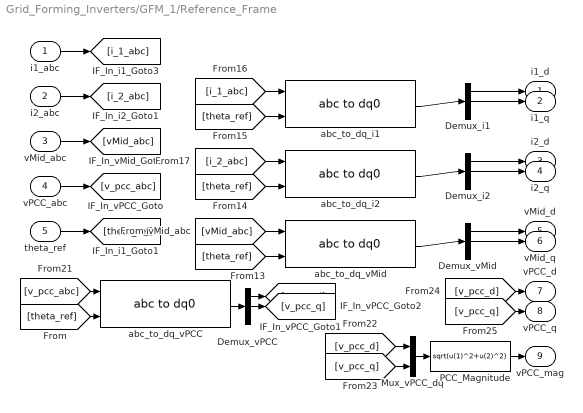
== system Grid_Forming_Inverters/GFM_1/Reference_Frame ==
  i1_abc : Inport
  i2_abc : Inport  Port=2
  vMid_abc : Inport  Port=3
  vPCC_abc : Inport  Port=4
  theta_ref : Inport  Port=5
  Demux_i1 : Demux  Outputs=3
  Demux_i2 : Demux  Outputs=3
  Demux_vMid : Demux  Outputs=3
  Demux_vPCC : Demux  Outputs=3
  Mux_vPCC_dq : Mux  Inputs=2
  PCC_Magnitude : Fcn  Expr=sqrt(u(1)^2+u(2)^2)
  abc_to_dq_i1 : spsabctodq0Lib/abc to dq0  Alignment=Aligned with phase A axis
  abc_to_dq_i2 : spsabctodq0Lib/abc to dq0  Alignment=Aligned with phase A axis
  abc_to_dq_vMid : spsabctodq0Lib/abc to dq0  Alignment=Aligned with phase A axis
  abc_to_dq_vPCC : spsabctodq0Lib/abc to dq0  Alignment=Aligned with phase A axis
  i1_d : Outport
  i1_q : Outport  Port=2
  i2_d : Outport  Port=3
  i2_q : Outport  Port=4
  vMid_d : Outport  Port=5
  vMid_q : Outport  Port=6
  vPCC_d : Outport  Port=7
  vPCC_q : Outport  Port=8
  vPCC_mag : Outport  Port=9
  wires:
  abc_to_dq_i1/1 -> Demux_i1/1
  Demux_i1/1 -> i1_d/1
  Demux_i1/2 -> i1_q/1
  abc_to_dq_i2/1 -> Demux_i2/1
  Demux_i2/1 -> i2_d/1
  Demux_i2/2 -> i2_q/1
  abc_to_dq_vMid/1 -> Demux_vMid/1
  Demux_vMid/1 -> vMid_d/1
  Demux_vMid/2 -> vMid_q/1
  abc_to_dq_vPCC/1 -> Demux_vPCC/1
  Mux_vPCC_dq/1 -> PCC_Magnitude/1
  PCC_Magnitude/1 -> vPCC_mag/1
  theta_ref/1 -> [theta_ref]
  [theta_ref] -> abc_to_dq_vPCC/2
  [theta_ref] -> abc_to_dq_vMid/2
  [theta_ref] -> abc_to_dq_i2/2
  [theta_ref] -> abc_to_dq_i1/2
  i1_abc/1 -> [i_1_abc]
  i2_abc/1 -> [i_2_abc]
  [i_1_abc] -> abc_to_dq_i1/1
  [i_2_abc] -> abc_to_dq_i2/1
  vPCC_abc/1 -> [v_pcc_abc]
  vMid_abc/1 -> [vMid_abc]
  [v_pcc_abc] -> abc_to_dq_vPCC/1
  Demux_vPCC/1 -> [v_pcc_d]
  Demux_vPCC/2 -> [v_pcc_q]
  [v_pcc_q] -> Mux_vPCC_dq/2
  [v_pcc_d] -> Mux_vPCC_dq/1
  [v_pcc_d] -> vPCC_d/1
  [v_pcc_q] -> vPCC_q/1
  [vMid_abc] -> abc_to_dq_vMid/1

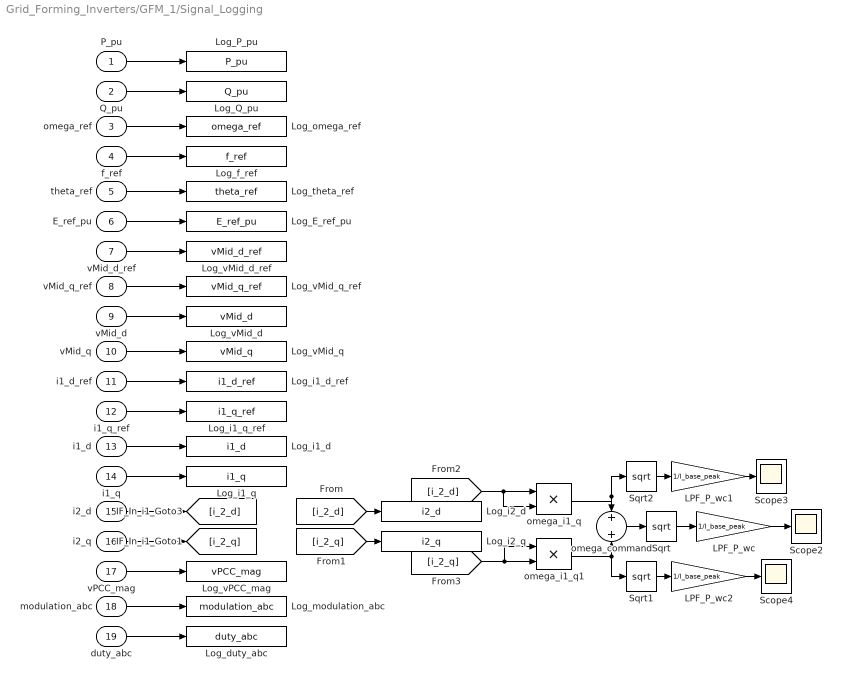
== system Grid_Forming_Inverters/GFM_1/Signal_Logging ==
  P_pu : Inport
  Q_pu : Inport  Port=2
  omega_ref : Inport  Port=3
  f_ref : Inport  Port=4
  theta_ref : Inport  Port=5
  E_ref_pu : Inport  Port=6
  vMid_d_ref : Inport  Port=7
  vMid_q_ref : Inport  Port=8
  vMid_d : Inport  Port=9
  vMid_q : Inport  Port=10
  i1_d_ref : Inport  Port=11
  i1_q_ref : Inport  Port=12
  i1_d : Inport  Port=13
  i1_q : Inport  Port=14
  i2_d : Inport  Port=15
  i2_q : Inport  Port=16
  vPCC_mag : Inport  Port=17
  modulation_abc : Inport  Port=18
  duty_abc : Inport  Port=19
  LPF_P_wc : Gain  Gain=1/I_base_peak
  LPF_P_wc1 : Gain  Gain=1/I_base_peak
  LPF_P_wc2 : Gain  Gain=1/I_base_peak
  Log_E_ref_pu : ToWorkspace  VariableName=E_ref_pu  SaveFormat=Timeseries  SampleTime=-1
  Log_P_pu : ToWorkspace  VariableName=P_pu  SaveFormat=Timeseries  SampleTime=-1
  Log_Q_pu : ToWorkspace  VariableName=Q_pu  SaveFormat=Timeseries  SampleTime=-1
  Log_duty_abc : ToWorkspace  VariableName=duty_abc  SaveFormat=Timeseries  SampleTime=-1
  Log_f_ref : ToWorkspace  VariableName=f_ref  SaveFormat=Timeseries  SampleTime=-1
  Log_i1_d : ToWorkspace  VariableName=i1_d  SaveFormat=Timeseries  SampleTime=-1
  Log_i1_d_ref : ToWorkspace  VariableName=i1_d_ref  SaveFormat=Timeseries  SampleTime=-1
  Log_i1_q : ToWorkspace  VariableName=i1_q  SaveFormat=Timeseries  SampleTime=-1
  Log_i1_q_ref : ToWorkspace  VariableName=i1_q_ref  SaveFormat=Timeseries  SampleTime=-1
  Log_i2_d : ToWorkspace  VariableName=i2_d  SaveFormat=Timeseries  SampleTime=-1
  Log_i2_q : ToWorkspace  VariableName=i2_q  SaveFormat=Timeseries  SampleTime=-1
  Log_modulation_abc : ToWorkspace  VariableName=modulation_abc  SaveFormat=Timeseries  SampleTime=-1
  Log_omega_ref : ToWorkspace  VariableName=omega_ref  SaveFormat=Timeseries  SampleTime=-1
  Log_theta_ref : ToWorkspace  VariableName=theta_ref  SaveFormat=Timeseries  SampleTime=-1
  Log_vMid_d : ToWorkspace  VariableName=vMid_d  SaveFormat=Timeseries  SampleTime=-1
  Log_vMid_d_ref : ToWorkspace  VariableName=vMid_d_ref  SaveFormat=Timeseries  SampleTime=-1
  Log_vMid_q : ToWorkspace  VariableName=vMid_q  SaveFormat=Timeseries  SampleTime=-1
  Log_vMid_q_ref : ToWorkspace  VariableName=vMid_q_ref  SaveFormat=Timeseries  SampleTime=-1
  Log_vPCC_mag : ToWorkspace  VariableName=vPCC_mag  SaveFormat=Timeseries  SampleTime=-1
  Scope2 : Scope
  Scope3 : Scope
  Scope4 : Scope
  Sqrt : Sqrt
  Sqrt1 : Sqrt
  Sqrt2 : Sqrt
  omega_command : Sum
  omega_i1_q : Product
  omega_i1_q1 : Product
  wires:
  P_pu/1 -> Log_P_pu/1
  Q_pu/1 -> Log_Q_pu/1
  omega_ref/1 -> Log_omega_ref/1
  f_ref/1 -> Log_f_ref/1
  theta_ref/1 -> Log_theta_ref/1
  E_ref_pu/1 -> Log_E_ref_pu/1
  vMid_d_ref/1 -> Log_vMid_d_ref/1
  vMid_q_ref/1 -> Log_vMid_q_ref/1
  vMid_d/1 -> Log_vMid_d/1
  vMid_q/1 -> Log_vMid_q/1
  i1_d_ref/1 -> Log_i1_d_ref/1
  i1_q_ref/1 -> Log_i1_q_ref/1
  i1_d/1 -> Log_i1_d/1
  i1_q/1 -> Log_i1_q/1
  i2_d/1 -> [i_2_d]
  vPCC_mag/1 -> Log_vPCC_mag/1
  modulation_abc/1 -> Log_modulation_abc/1
  duty_abc/1 -> Log_duty_abc/1
  [i_2_d] -> Log_i2_d/1
  i2_q/1 -> [i_2_q]
  [i_2_q] -> Log_i2_q/1
  [i_2_d] -> omega_i1_q/2, omega_i1_q/1
  [i_2_q] -> omega_i1_q1/1, omega_i1_q1/2
  omega_i1_q/1 -> Sqrt2/1, omega_command/1
  omega_i1_q1/1 -> Sqrt1/1, omega_command/2
  omega_command/1 -> Sqrt/1
  Sqrt/1 -> LPF_P_wc/1
  LPF_P_wc/1 -> Scope2/1
  Sqrt2/1 -> LPF_P_wc1/1
  LPF_P_wc1/1 -> Scope3/1
  Sqrt1/1 -> LPF_P_wc2/1
  LPF_P_wc2/1 -> Scope4/1

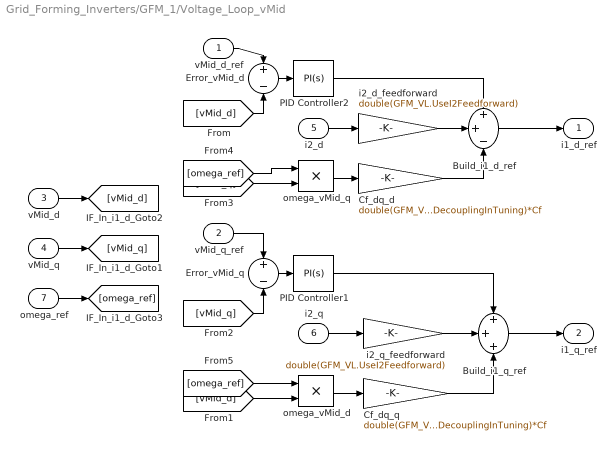
== system Grid_Forming_Inverters/GFM_1/Voltage_Loop_vMid ==
  vMid_d_ref : Inport
  vMid_q_ref : Inport  Port=2
  vMid_d : Inport  Port=3
  vMid_q : Inport  Port=4
  i2_d : Inport  Port=5
  i2_q : Inport  Port=6
  omega_ref : Inport  Port=7
  Build_i1_d_ref : Sum  Inputs=++-
  Build_i1_q_ref : Sum  Inputs=+++
  Cf_dq_d : Gain  Gain=double(GFM_VL.UseDQDecouplingInTuning)*Cf
  Cf_dq_q : Gain  Gain=double(GFM_VL.UseDQDecouplingInTuning)*Cf
  Error_vMid_d : Sum  Inputs=+-
  Error_vMid_q : Sum  Inputs=+-
  PID Controller1 : slpidlib/PID Controller  Controller=PI  Form=Parallel  TimeDomain=Continuous-time  UseExternalTs=off  SampleTime=-1  IntegratorMethod=Forward Euler  FilterMethod=Forward Euler  ControllerParametersSource=internal  P=GFM_VL.Kp  I=GFM_VL.Ki  UseKiTs=off  D=0  UseExternalDerivativeSource=off  N=100  UseFilter=on  TunerSelectOption=Transfer Function Based (PID Tuner App)  InitialConditionSource=internal  InitialConditionForIntegrator=0  InitialConditionForFilter=0  DifferentiatorICPrevScaledInput=0  ExternalReset=none  TrackingMode=off  Kt=1  LimitOutput=off  SatLimitsSource=internal  UpperSaturationLimit=inf  LowerSaturationLimit=-inf  LinearizeAsGain=on  AntiWindupMode=none  Kb=1  LimitIntegrator=off  UpperIntegratorSaturationLimit=inf  LowerIntegratorSaturationLimit=-inf  POutMin=[]  POutMax=[]  IOutMin=[]  IOutMax=[]  DOutMin=[]  DOutMax=[]  NOutMin=[]  NOutMax=[]  SumOutMin=[]  SumOutMax=[]  SaturationOutMin=[]  SaturationOutMax=[]  PParamMin=[]  PParamMax=[]  IParamMin=[]  IParamMax=[]  DParamMin=[]  DParamMax=[]  NParamMin=[]  NParamMax=[]  KbParamMin=[]  KbParamMax=[]  KtParamMin=[]  KtParamMax=[]  KbOutMin=[]  KbOutMax=[]  KtOutMin=[]  KtOutMax=[]  IntegratorOutMin=[]  IntegratorOutMax=[]  FilterOutMin=[]  FilterOutMax=[]  SumI1OutMin=[]  SumI1OutMax=[]  SumI2OutMin=[]  SumI2OutMax=[]  SumI3OutMin=[]  SumI3OutMax=[]  SumI4OutMin=[]  SumI4OutMax=[]  SumDOutMin=[]  SumDOutMax=[]  DifferentiatorOutMin=[]  DifferentiatorOutMax=[]  FilterDiffOutCoefMin=[]  FilterDiffOutCoefMax=[]  ReciprocalOutMin=[]  ReciprocalOutMax=[]  SumDenOutMin=[]  SumDenOutMax=[]  SumNumOutMin=[]  SumNumOutMax=[]  DivideOutMin=[]  DivideOutMax=[]  UdiffTsProdOutMin=[]  UdiffTsProdOutMax=[]  NTsProdOutMin=[]  NTsProdOutMax=[]  UintegralTsProdOutMin=[]  UintegralTsProdOutMax=[]  UngainTsProdOutMin=[]  UngainTsProdOutMax=[]  ClampingZeroOutDataTypeStr=Inherit: Inherit via back propagation  ClampingZeroOutMin=[]  ClampingZeroOutMax=[]  FilterDenConstantOutDataTypeStr=Inherit: Inherit via back propagation  FilterDenConstantOutMin=[]  FilterDenConstantOutMax=[]  PCopyOutDataTypeStr=Inherit: Inherit via back propagation  PCopyOutMin=[]  PCopyOutMax=[]  NCopyOutDataTypeStr=Inherit: Inherit via back propagation  NCopyOutMin=[]  NCopyOutMax=[]  IntegratorContinuousStateAttributes=''  IntegratorStateMustResolveToSignalObject=off  IntegratorRTWStateStorageClass=Auto  FilterContinuousStateAttributes=''  FilterStateMustResolveToSignalObject=off  FilterRTWStateStorageClass=Auto  ParallelPVariant=InternalParameters  IdealPVariant=Disabled  IVariant=InternalParameters  DVariant=Disabled  IntegratorVariant=Continuous  SatVariant=Disabled  AWVariant=Passthrough  PCopyVariant=Disabled  TRVariant=Disabled  FdbkBlocksVariant=Forward  IdealPFdbkVariant=Disabled  SatFdbkVariant=Disabled  DerivativeFilterVariant=Disabled  NVariant=Disabled  NCopyVariant=Disabled_SignalSpec  FilterICVariant=Disabled  IntegratorICVariant=InternalICs  ExternalResetVariant=Disabled  TRSumVariant=Passthrough  SumFdbkVariant=Disabled  SumVariant=Sum_PI  TsampFilterVariant=InternalTs  TsampNgainVariant=Passthrough  TsampIntegralVariant=Disabled_SignalSpec  ExternalSaturationOutDataTypeStr=Inherit: Same as second input  DerivativeSourceVariant=Disabled  PreIntVariant=InternalPreInt
  PID Controller2 : slpidlib/PID Controller  Controller=PI  Form=Parallel  TimeDomain=Continuous-time  UseExternalTs=off  SampleTime=-1  IntegratorMethod=Forward Euler  FilterMethod=Forward Euler  ControllerParametersSource=internal  P=GFM_VL.Kp  I=GFM_VL.Ki  UseKiTs=off  D=0  UseExternalDerivativeSource=off  N=100  UseFilter=on  TunerSelectOption=Transfer Function Based (PID Tuner App)  InitialConditionSource=internal  InitialConditionForIntegrator=0  InitialConditionForFilter=0  DifferentiatorICPrevScaledInput=0  ExternalReset=none  TrackingMode=off  Kt=1  LimitOutput=off  SatLimitsSource=internal  UpperSaturationLimit=inf  LowerSaturationLimit=-inf  LinearizeAsGain=on  AntiWindupMode=none  Kb=1  LimitIntegrator=off  UpperIntegratorSaturationLimit=inf  LowerIntegratorSaturationLimit=-inf  POutMin=[]  POutMax=[]  IOutMin=[]  IOutMax=[]  DOutMin=[]  DOutMax=[]  NOutMin=[]  NOutMax=[]  SumOutMin=[]  SumOutMax=[]  SaturationOutMin=[]  SaturationOutMax=[]  PParamMin=[]  PParamMax=[]  IParamMin=[]  IParamMax=[]  DParamMin=[]  DParamMax=[]  NParamMin=[]  NParamMax=[]  KbParamMin=[]  KbParamMax=[]  KtParamMin=[]  KtParamMax=[]  KbOutMin=[]  KbOutMax=[]  KtOutMin=[]  KtOutMax=[]  IntegratorOutMin=[]  IntegratorOutMax=[]  FilterOutMin=[]  FilterOutMax=[]  SumI1OutMin=[]  SumI1OutMax=[]  SumI2OutMin=[]  SumI2OutMax=[]  SumI3OutMin=[]  SumI3OutMax=[]  SumI4OutMin=[]  SumI4OutMax=[]  SumDOutMin=[]  SumDOutMax=[]  DifferentiatorOutMin=[]  DifferentiatorOutMax=[]  FilterDiffOutCoefMin=[]  FilterDiffOutCoefMax=[]  ReciprocalOutMin=[]  ReciprocalOutMax=[]  SumDenOutMin=[]  SumDenOutMax=[]  SumNumOutMin=[]  SumNumOutMax=[]  DivideOutMin=[]  DivideOutMax=[]  UdiffTsProdOutMin=[]  UdiffTsProdOutMax=[]  NTsProdOutMin=[]  NTsProdOutMax=[]  UintegralTsProdOutMin=[]  UintegralTsProdOutMax=[]  UngainTsProdOutMin=[]  UngainTsProdOutMax=[]  ClampingZeroOutDataTypeStr=Inherit: Inherit via back propagation  ClampingZeroOutMin=[]  ClampingZeroOutMax=[]  FilterDenConstantOutDataTypeStr=Inherit: Inherit via back propagation  FilterDenConstantOutMin=[]  FilterDenConstantOutMax=[]  PCopyOutDataTypeStr=Inherit: Inherit via back propagation  PCopyOutMin=[]  PCopyOutMax=[]  NCopyOutDataTypeStr=Inherit: Inherit via back propagation  NCopyOutMin=[]  NCopyOutMax=[]  IntegratorContinuousStateAttributes=''  IntegratorStateMustResolveToSignalObject=off  IntegratorRTWStateStorageClass=Auto  FilterContinuousStateAttributes=''  FilterStateMustResolveToSignalObject=off  FilterRTWStateStorageClass=Auto  ParallelPVariant=InternalParameters  IdealPVariant=Disabled  IVariant=InternalParameters  DVariant=Disabled  IntegratorVariant=Continuous  SatVariant=Disabled  AWVariant=Passthrough  PCopyVariant=Disabled  TRVariant=Disabled  FdbkBlocksVariant=Forward  IdealPFdbkVariant=Disabled  SatFdbkVariant=Disabled  DerivativeFilterVariant=Disabled  NVariant=Disabled  NCopyVariant=Disabled_SignalSpec  FilterICVariant=Disabled  IntegratorICVariant=InternalICs  ExternalResetVariant=Disabled  TRSumVariant=Passthrough  SumFdbkVariant=Disabled  SumVariant=Sum_PI  TsampFilterVariant=InternalTs  TsampNgainVariant=Passthrough  TsampIntegralVariant=Disabled_SignalSpec  ExternalSaturationOutDataTypeStr=Inherit: Same as second input  DerivativeSourceVariant=Disabled  PreIntVariant=InternalPreInt
  i2_d_feedforward : Gain  Gain=double(GFM_VL.UseI2Feedforward)
  i2_q_feedforward : Gain  Gain=double(GFM_VL.UseI2Feedforward)
  omega_vMid_d : Product
  omega_vMid_q : Product
  i1_d_ref : Outport
  i1_q_ref : Outport  Port=2
  wires:
  vMid_d_ref/1 -> Error_vMid_d/1
  vMid_q_ref/1 -> Error_vMid_q/1
  i2_d/1 -> i2_d_feedforward/1
  i2_q/1 -> i2_q_feedforward/1
  omega_vMid_q/1 -> Cf_dq_d/1
  omega_vMid_d/1 -> Cf_dq_q/1
  PID Controller2/1 -> Build_i1_d_ref/1
  i2_d_feedforward/1 -> Build_i1_d_ref/2
  Cf_dq_d/1 -> Build_i1_d_ref/3
  i2_q_feedforward/1 -> Build_i1_q_ref/2
  Cf_dq_q/1 -> Build_i1_q_ref/3
  Build_i1_d_ref/1 -> i1_d_ref/1
  Build_i1_q_ref/1 -> i1_q_ref/1
  vMid_d/1 -> [vMid_d]
  [vMid_d] -> Error_vMid_d/2
  [vMid_d] -> omega_vMid_d/2
  Error_vMid_d/1 -> PID Controller2/1
  vMid_q/1 -> [vMid_q]
  [vMid_q] -> Error_vMid_q/2
  [vMid_q] -> omega_vMid_q/2
  omega_ref/1 -> [omega_ref]
  [omega_ref] -> omega_vMid_q/1
  [omega_ref] -> omega_vMid_d/1
  Error_vMid_q/1 -> PID Controller1/1
  PID Controller1/1 -> Build_i1_q_ref/1
